simulink model "sem_harmonic_mdl"  (R2020b)
settings: Solver=ode15s  StartTime=0.0  StopTime=10  RelTol=1e-3
settings Model: PauseTimes=1  Creator=Arsen  LastModifiedBy=Arsen
settings DebuggingCC: UnderSpecifiedDimensionMsg=warning

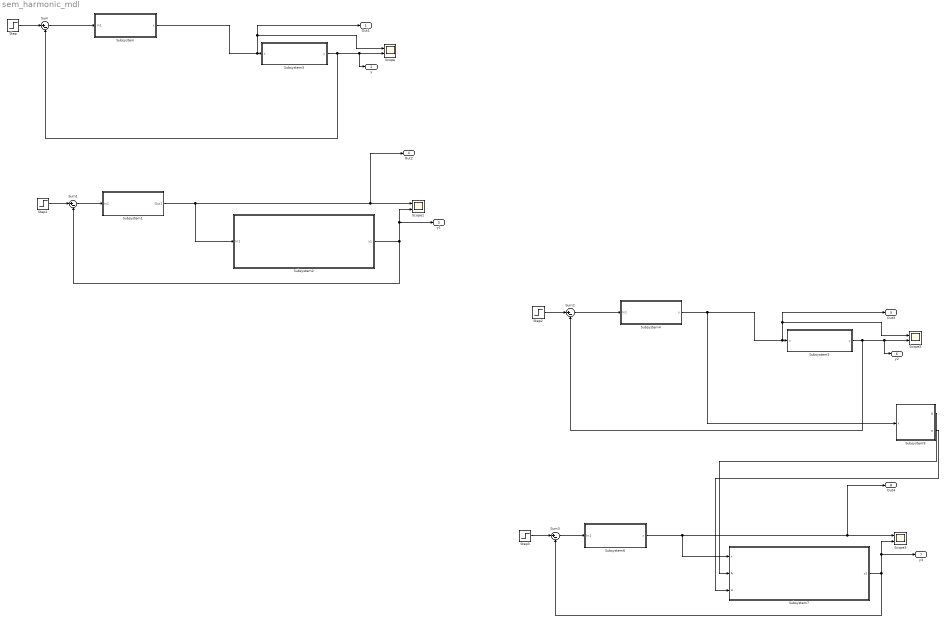
== system sem_harmonic_mdl ==
  Scope{,1..3} (4 alike) : Scope  NumInputPorts=2
  Step{,1..3} (4 alike) : Step  Time=0  After=0  SampleTime=0
  Subsystem : Subsystem
  Subsystem1 : Subsystem
  Subsystem2 : Subsystem
  Subsystem3 : Subsystem
  Subsystem4 : Subsystem
  Subsystem5 : Subsystem
  Subsystem6 : Subsystem
  Subsystem7 : Subsystem
  Subsystem9 : Subsystem
  Sum{,1..3} (4 alike) : Sum  Inputs=|+-
  Out1 : Outport
  y : Outport  Port=2
  y1 : Outport  Port=3
  Out2 : Outport  Port=4
  Out3 : Outport  Port=5
  y2 : Outport  Port=6
  y3 : Outport  Port=7
  Out4 : Outport  Port=8
  wires:
  Step/1 -> Sum/1
  Step1/1 -> Sum1/1
  Subsystem/1(x) -> Scope/1, Out1/1, Subsystem3/1(x)
  Sum/1 -> Subsystem/1(In1)
  Sum1/1 -> Subsystem1/1(In1)
  Subsystem2/1(y1) -> y1/1, Scope1/2, Sum1/2
  Subsystem3/1(y) -> Sum/2, Scope/2, y/1
  Subsystem1/1(Out1) -> Subsystem2/1(In1), Out2/1, Scope1/1
  Sum3/1 -> Subsystem6/1(In1)
  Subsystem6/1(x) -> Subsystem7/1(x), Scope3/1, Out4/1
  Subsystem9/1(A) -> Subsystem7/2(A)
  Subsystem9/2(w) -> Subsystem7/3(w)
  Subsystem4/1(x) -> Subsystem9/1(x), Scope2/1, Out3/1, Subsystem5/1(x)
  Subsystem7/1(y1) -> y3/1, Scope3/2, Sum3/2
  Sum2/1 -> Subsystem4/1(In1)
  Subsystem5/1(y) -> Sum2/2, Scope2/2, y2/1
  Step2/1 -> Sum2/1
  Step3/1 -> Sum3/1

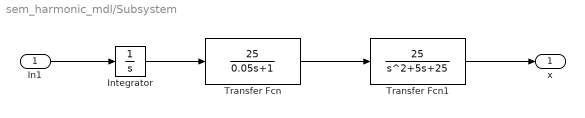
== system sem_harmonic_mdl/Subsystem ==
  In1 : Inport
  Integrator : Integrator  InitialCondition=1
  Transfer Fcn : TransferFcn  Numerator=[25]  Denominator=[0.05 1]
  Transfer Fcn1 : TransferFcn  Numerator=[25]  Denominator=[1 5 25]
  x : Outport
  wires:
  Integrator/1 -> Transfer Fcn/1
  Transfer Fcn/1 -> Transfer Fcn1/1
  In1/1 -> Integrator/1
  Transfer Fcn1/1 -> x/1

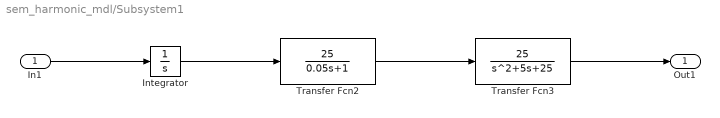
== system sem_harmonic_mdl/Subsystem1 ==
  In1 : Inport
  Integrator : Integrator  InitialCondition=1
  Transfer Fcn2 : TransferFcn  Numerator=[25]  Denominator=[0.05 1]
  Transfer Fcn3 : TransferFcn  Numerator=[25]  Denominator=[1 5 25]
  Out1 : Outport
  wires:
  Transfer Fcn2/1 -> Transfer Fcn3/1
  Integrator/1 -> Transfer Fcn2/1
  In1/1 -> Integrator/1
  Transfer Fcn3/1 -> Out1/1

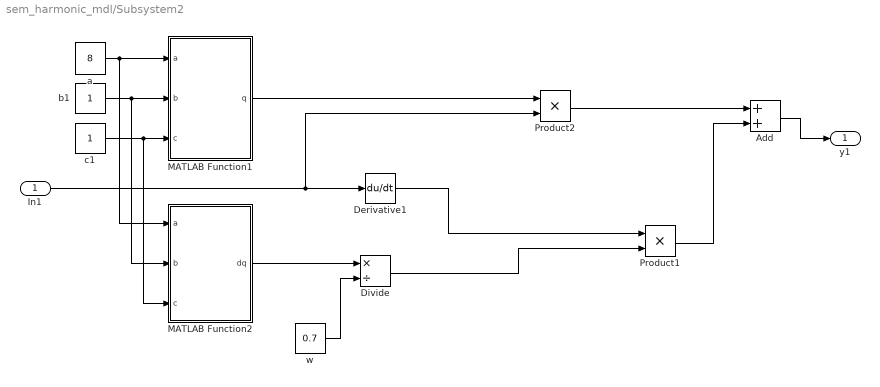
== system sem_harmonic_mdl/Subsystem2 ==
  In1 : Inport
  Add : Sum
  Derivative1 : Derivative
  Divide : Product  Inputs=*/
  MATLAB Function1 : MATLAB Function  TreatAsAtomicUnit=on
  MATLAB Function2 : MATLAB Function  TreatAsAtomicUnit=on
  Product1 : Product
  Product2 : Product
  a : Constant  Value=8
  b1 : Constant
  c1 : Constant
  w : Constant  Value=0.7
  y1 : Outport
  wires:
  w/1 -> Divide/2
  b1/1 -> MATLAB Function2/2(b), MATLAB Function1/2(b)
  MATLAB Function2/1(dq) -> Divide/1
  c1/1 -> MATLAB Function2/3(c), MATLAB Function1/3(c)
  Derivative1/1 -> Product1/1
  Product1/1 -> Add/2
  In1/1 -> Product2/2, Derivative1/1
  Divide/1 -> Product1/2
  a/1 -> MATLAB Function2/1(a), MATLAB Function1/1(a)
  Add/1 -> y1/1
  MATLAB Function1/1(q) -> Product2/1
  Product2/1 -> Add/1

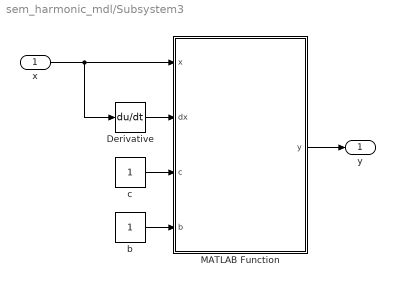
== system sem_harmonic_mdl/Subsystem3 ==
  x : Inport
  Derivative : Derivative
  MATLAB Function : MATLAB Function  TreatAsAtomicUnit=on
  b : Constant
  c : Constant
  y : Outport
  wires:
  c/1 -> MATLAB Function/3(c)
  MATLAB Function/1(y) -> y/1
  Derivative/1 -> MATLAB Function/2(dx)
  b/1 -> MATLAB Function/4(b)
  x/1 -> Derivative/1, MATLAB Function/1(x)

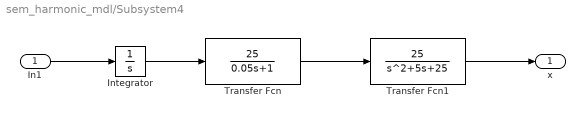
== system sem_harmonic_mdl/Subsystem4 ==
  In1 : Inport
  Integrator : Integrator  InitialCondition=1
  Transfer Fcn : TransferFcn  Numerator=[25]  Denominator=[0.05 1]
  Transfer Fcn1 : TransferFcn  Numerator=[25]  Denominator=[1 5 25]
  x : Outport
  wires:
  Integrator/1 -> Transfer Fcn/1
  Transfer Fcn/1 -> Transfer Fcn1/1
  In1/1 -> Integrator/1
  Transfer Fcn1/1 -> x/1

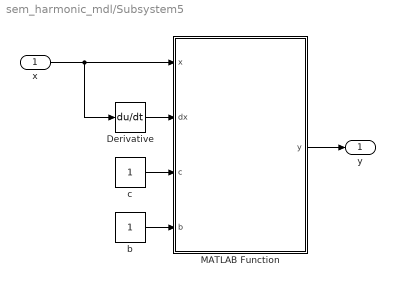
== system sem_harmonic_mdl/Subsystem5 ==
  x : Inport
  Derivative : Derivative
  MATLAB Function : MATLAB Function  TreatAsAtomicUnit=on
  b : Constant
  c : Constant
  y : Outport
  wires:
  c/1 -> MATLAB Function/3(c)
  MATLAB Function/1(y) -> y/1
  Derivative/1 -> MATLAB Function/2(dx)
  b/1 -> MATLAB Function/4(b)
  x/1 -> Derivative/1, MATLAB Function/1(x)

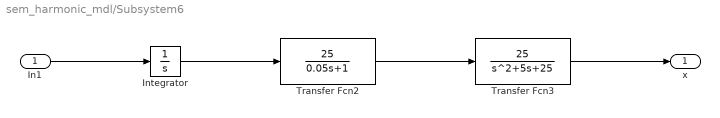
== system sem_harmonic_mdl/Subsystem6 ==
  In1 : Inport
  Integrator : Integrator  InitialCondition=1
  Transfer Fcn2 : TransferFcn  Numerator=[25]  Denominator=[0.05 1]
  Transfer Fcn3 : TransferFcn  Numerator=[25]  Denominator=[1 5 25]
  x : Outport
  wires:
  Transfer Fcn2/1 -> Transfer Fcn3/1
  Integrator/1 -> Transfer Fcn2/1
  In1/1 -> Integrator/1
  Transfer Fcn3/1 -> x/1

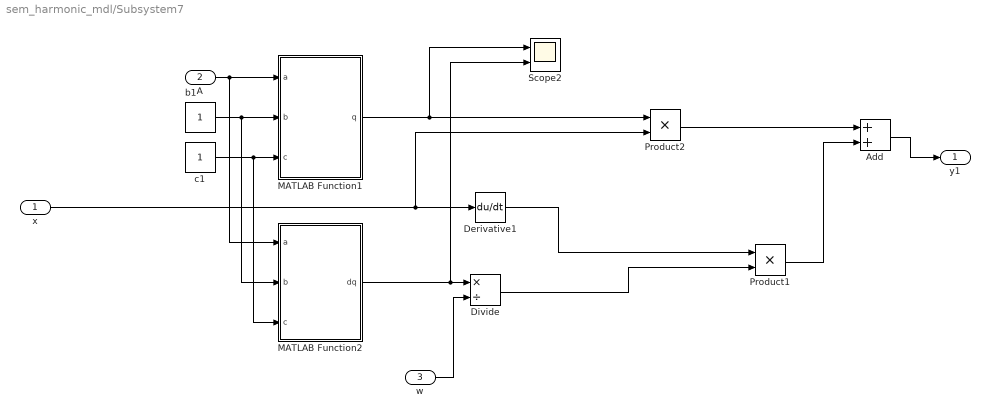
== system sem_harmonic_mdl/Subsystem7 ==
  x : Inport
  A : Inport  Port=2
  w : Inport  Port=3
  Add : Sum
  Derivative1 : Derivative
  Divide : Product  Inputs=*/
  MATLAB Function1 : MATLAB Function  TreatAsAtomicUnit=on
  MATLAB Function2 : MATLAB Function  TreatAsAtomicUnit=on
  Product1 : Product
  Product2 : Product
  Scope2 : Scope  NumInputPorts=2
  b1 : Constant
  c1 : Constant
  y1 : Outport
  wires:
  b1/1 -> MATLAB Function2/2(b), MATLAB Function1/2(b)
  MATLAB Function2/1(dq) -> Scope2/2, Divide/1
  c1/1 -> MATLAB Function2/3(c), MATLAB Function1/3(c)
  Derivative1/1 -> Product1/1
  Product1/1 -> Add/2
  x/1 -> Product2/2, Derivative1/1
  Divide/1 -> Product1/2
  A/1 -> MATLAB Function2/1(a), MATLAB Function1/1(a)
  Add/1 -> y1/1
  MATLAB Function1/1(q) -> Scope2/1, Product2/1
  Product2/1 -> Add/1
  w/1 -> Divide/2

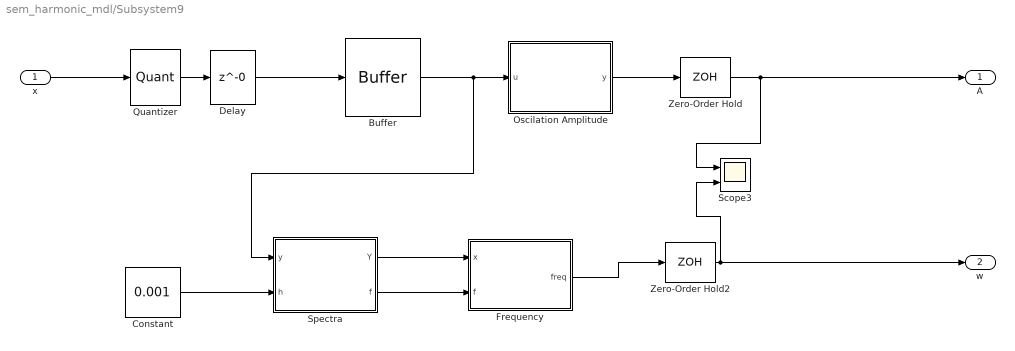
== system sem_harmonic_mdl/Subsystem9 ==
  x : Inport
  Buffer : Buffer  N=2000  V=1500  OutputFrames=off
  Constant : Constant  Value=0.001
  Delay : Delay  DelayLength=0  InitialCondition=0  SampleTime=0.001
  Frequency : MATLAB Function  TreatAsAtomicUnit=on
  Oscilation Amplitude : MATLAB Function  TreatAsAtomicUnit=on
  Quantizer : Quantizer  QuantizationInterval=0.001
  Scope3 : Scope  NumInputPorts=2
  Spectra : MATLAB Function  TreatAsAtomicUnit=on
  Zero-Order Hold : ZeroOrderHold  SampleTime=-1
  Zero-Order Hold2 : ZeroOrderHold  SampleTime=-1
  A : Outport
  w : Outport  Port=2
  wires:
  Constant/1 -> Spectra/2(h)
  x/1 -> Quantizer/1
  Delay/1 -> Buffer/1
  Frequency/1(freq) -> Zero-Order Hold2/1
  Spectra/1(Y) -> Frequency/1(x)
  Quantizer/1 -> Delay/1
  Oscilation Amplitude/1(y) -> Zero-Order Hold/1
  Spectra/2(f) -> Frequency/2(f)
  Buffer/1 -> Spectra/1(y), Oscilation Amplitude/1("u ")
  Zero-Order Hold/1 -> Scope3/1, A/1
  Zero-Order Hold2/1 -> Scope3/2, w/1

== matlab function sem_harmonic_mdl/Subsystem2/MATLAB Function1 ==
  data: a input; b input; q output; c input
function q = fcn(a, b, c)
    q = 4*c/(pi*a)*sqrt(1-b^2/a^2);
end

== matlab function sem_harmonic_mdl/Subsystem3/MATLAB Function ==
  data: x input; dx input; y output; c input; b input
function y = fcn(x, dx, c, b)
    if dx>=0
        if (x >= b)
            y = c;
        else
            y = -c;
        end
    else
        if (x > -b)
            y = c;
        else
            y = -c;
        end
    end
end

== matlab function sem_harmonic_mdl/Subsystem2/MATLAB Function2 ==
  data: a input; b input; dq output; c input
function dq = fcn(a, b, c)
    
    dq = 4*c*b/(pi*a^2);

end

== matlab function sem_harmonic_mdl/Subsystem5/MATLAB Function ==
  data: x input; dx input; y output; c input; b input
function y = fcn(x, dx, c, b)
    if dx>=0
        if (x >= b)
            y = c;
        else
            y = -c;
        end
    else
        if (x > -b)
            y = c;
        else
            y = -c;
        end
    end
end

== matlab function sem_harmonic_mdl/Subsystem7/MATLAB Function1 ==
  data: a input; b input; q output; c input
function q = fcn(a, b, c)
    
    if a < b
        q = 0;
    else
        q = 4*c/(pi*a)*sqrt(1-b^2/a^2);
    end
end

== matlab function sem_harmonic_mdl/Subsystem7/MATLAB Function2 ==
  data: a input; b input; dq output; c input
function dq = fcn(a, b, c)
    
    if a < b
        dq = 0;
    else
         dq = -4*c*b/(pi*a^2);
    end
   
end

== matlab function sem_harmonic_mdl/Subsystem9/Frequency ==
  data: x input; freq output; f input
function freq = fcn(x, f)
[~, i] = max(x);
freq = f(i) * 2 * pi;
    if freq == 0
        freq = 1;
    end
end

== matlab function sem_harmonic_mdl/Subsystem9/Oscilation Amplitude ==
  data: u input; y output
function y = fcn(u)
    y = (max(u)-min(u))/2;
%     if y < 1
%         y = 1.001;
%     end
end

== matlab function sem_harmonic_mdl/Subsystem9/Spectra ==
  data: y input; Y output; f output; h input
function [Y, f] = lab_spectra(y, h)
% x = x - mean (x);
% x = x.*tukeywin(length(x), 0.1);
% X1 = fft(x, length(x));
% X1 = abs (X1)/length(X1);
% X = X1(1: (length(X1)/2));
% X(2:length(x)/2) = x (2:length (x) /2)*2;
% f = (1/h)*(0:1:length(x)/2-1)/ length(x);
y = y - mean(y);
y = y.*tukeywin(length(y), 0.1);
Y1 = fft(y, length(y));
Y1 = abs(Y1)/length(Y1);
Y = Y1(1:(length(Y1)/2));
Y(2:length(y)/2) = Y(2:length(y)/2)*2;
f = (1/h)*(0:1:length(y)/2-1)/length(y);
end
